simulink model "T11_Sim_BPSK_2"  (R2015a)
settings: Solver=ode45  StartTime=0.0  StopTime=50  RelTol=1e-3
libraries: commdigbbndpm3 x2, commchan3 x1, commrandsrc2 x1
settings Model: Creator=User  LastModifiedBy=User

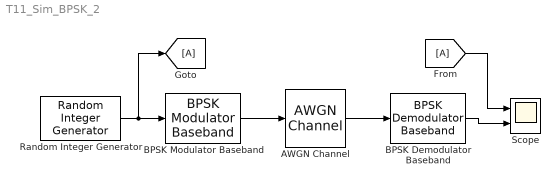
== system T11_Sim_BPSK_2 ==
  AWGN Channel : commchan3/AWGN Channel  InputProcessing=Columns as channels (frame based)  seed=67  noiseMode="Signal to noise ratio  (Eb/No)"  EbNodB=-10  EsNodB=4  SNRdB=10  bitsPerSym=1  Ps=1  Tsym=1  variance=1
  BPSK Demodulator Baseband : commdigbbndpm3/BPSK Demodulator Baseband  Ph=0  DecType=Hard decision  VarSource=Dialog  Variance=1  outDtype=Inherit via internal rule  derotateFactorWordLen=16
  BPSK Modulator Baseband : commdigbbndpm3/BPSK Modulator Baseband  Ph=0  outDtype=double  outWordLen=16  outUDDataType=sfix(16)  outFracLenMode=Best precision  outFracLen=15
  Random Integer Generator : commrandsrc2/Random Integer Generator  mul=2  seed=37  Ts=1  frameBased=off  sampPerFrame=1000  orient=off  outDataType=boolean
  Scope : Scope  NumInputPorts=2
      settings: YMin=-0.125~-0.125  YMax=1.125~1.125
  wires:
  Random Integer Generator/1 -> [A], BPSK Modulator Baseband/1
  BPSK Modulator Baseband/1 -> AWGN Channel/1
  AWGN Channel/1 -> BPSK Demodulator Baseband/1
  BPSK Demodulator Baseband/1 -> Scope/2
  [A] -> Scope/1
